simulink model "a_openloop"  (R2022b)
settings: Solver=VariableStepAuto  StartTime=0.0  StopTime=1.0  RelTol=1e-3
libraries: simulink x3, spsDCVoltageSourceLib x1, spsGroundLib x1, spsPermanentMagnetSynchronousMachineLib x1, spsThreePhaseVIMeasurementLib x1, spsUniversalBridgeLib x1, spspowerguiLib x1, sps_lib x1
settings Model: Creator=15403  LastModifiedBy=15403

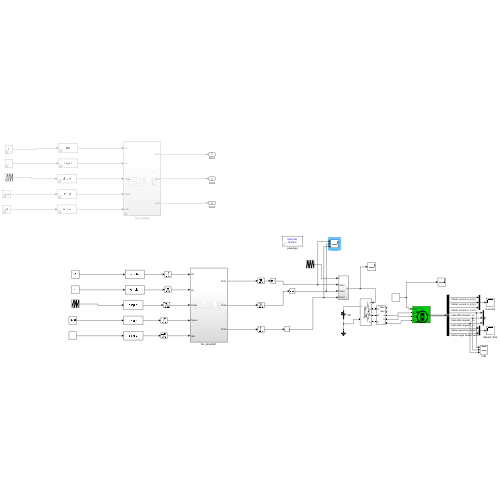
[thumbnail: Simulink's stored preview of the top-level diagram]
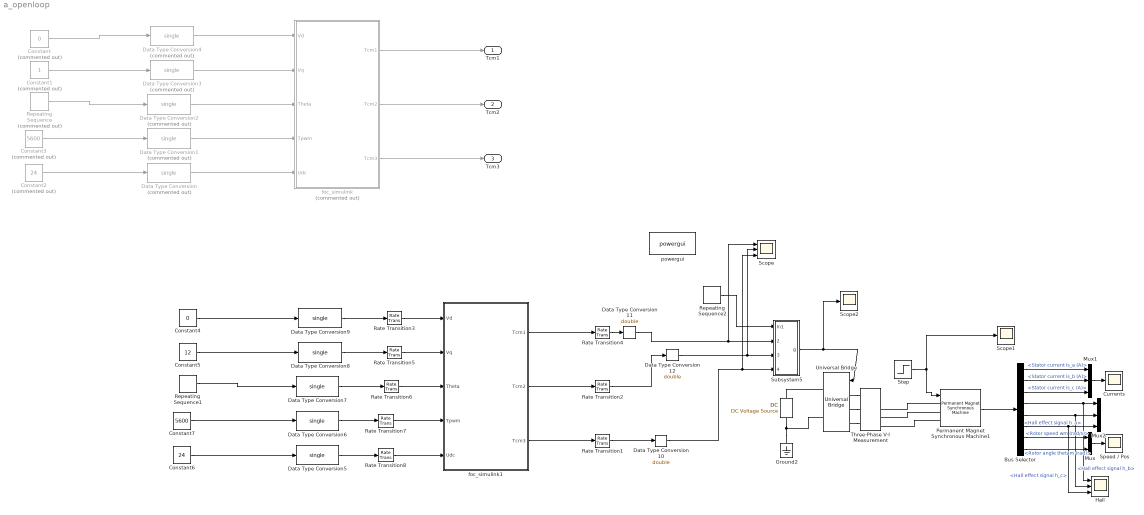
== system a_openloop ==
  Bus Selector : BusSelector  OutputSignals=Stator current is_a (A),Stator current is_b (A),Stator current is_c (A),Hall effect signal h_a,Hall effect signal h_b,Hall effect signal h_c,Rotor speed wm (rad/s),Rotor angle thetam (rad)
  Constant : Constant  Commented=on  Value=0
  Constant1 : Constant  Commented=on
  Constant2 : Constant  Commented=on  Value=24
  Constant3 : Constant  Commented=on  Value=5600
  Constant4 : Constant  Value=0
  Constant5 : Constant  Value=12
  Constant6 : Constant  Value=24
  Constant7 : Constant  Value=5600
  Currents : Scope
  "DC " : spsDCVoltageSourceLib/DC Voltage Source  Amplitude=24  Measurements=None
  Data Type Conversion{,1..4} (5 alike) : DataTypeConversion  Commented=on  OutDataTypeStr=single  SaturateOnIntegerOverflow=off  RndMeth=Floor
  Data Type Conversion10 : DataTypeConversion  OutDataTypeStr=double  SaturateOnIntegerOverflow=off  RndMeth=Floor
  Data Type Conversion11 : DataTypeConversion  OutDataTypeStr=double  SaturateOnIntegerOverflow=off  RndMeth=Floor
  Data Type Conversion12 : DataTypeConversion  OutDataTypeStr=double  SaturateOnIntegerOverflow=off  RndMeth=Floor
  Data Type Conversion{5..9} (5 alike) : DataTypeConversion  OutDataTypeStr=single  SaturateOnIntegerOverflow=off  RndMeth=Floor
  Ground2 : spsGroundLib/Ground  LConnTagsString=a
  Hall : Scope  NumInputPorts=3
  Mux : Mux  Inputs=2
  Mux1 : Mux  Inputs=3
  Mux2 : Mux  Inputs=3
  Permanent Magnet Synchronous Machine1 : spsPermanentMagnetSynchronousMachineLib/Permanent Magnet Synchronous Machine  NbPhases=3  FluxDistribution=Sinusoidal  RotorType=Round  MechanicalLoad=Torque Tm  PresetModel=No  ShowDetailedParameters=on  MeasurementBus=off  Resistance=0.6  Inductance=8.5e-3  dqInductances=[8.5e-3, 8.5e-3]  La=1.4e-3  MachineConstant=Flux linkage established by magnets (V.s)  Flux=0.034182  VoltageCst=6.1999  TorqueCst=0.051273  Flat=120  Mechanical=[1.1e-5,1e-4,1,0.02]  PolePairs=4  InitialConditions=[0,0, 0,0]  InitialConditions5ph=[0 0 0 0 0 0]  RefAngle=Aligned with phase A axis (original Park)  IterativeDiscreteModel=Trapezoidal non iterative  TsBlock=-1  TsPowergui=0
  Rate Transition{1..8} (8 alike) : RateTransition
  Repeating Sequence : simulink/Sources/Repeating Sequence  Commented=on  rep_seq_t=[0 0.1]  rep_seq_y=[0 2 * pi]
  Repeating Sequence1 : simulink/Sources/Repeating Sequence  rep_seq_t=[0 0.1]  rep_seq_y=[0 2 * pi]
  Repeating Sequence2 : simulink/Sources/Repeating Sequence  rep_seq_t=[0 1/15000 2/15000]  rep_seq_y=[0 2800 0]
  Scope : Scope  NumInputPorts=3
  Scope1 : Scope
  Scope2 : Scope
  Speed / Pos : Scope
  Step : Step  Time=0  After=0  SampleTime=0
  Subsystem5 : Subsystem
  Three-Phase V-I Measurement : spsThreePhaseVIMeasurementLib/Three-Phase V-I Measurement  VoltageMeasurement=phase-to-ground  SetLabelV=off  LabelV=Vabc  Vpu=off  VpuLL=off  CurrentMeasurement=yes  SetLabelI=off  LabelI=Iabc  Ipu=off  Pbase=100e6  Vbase=500e3  OutputType=Complex  PhasorSimulation=off  PSBequivalent=0
  Universal Bridge : spsUniversalBridgeLib/Universal Bridge  Arms=3  SnubberResistance=1e5  SnubberCapacitance=inf  Device=IGBT / Diodes  Ron=1e-3  Lon=0  ForwardVoltages="[  0  0  ]"  ForwardVoltage=0  GTOparameters=[ 10e-6 , 20e-6 ]  IGBTparameters=[ 1e-6 , 2e-6 ]  Measurements=None  Measurements_2=None  converterType=Rectifier
  foc_simulink : Subsystem  Commented=on
  foc_simulink1 : Subsystem
  powergui : sps_lib/powergui  Priority=1  SimulationMode=Discrete  SampleTime=0.000001  frequency=60  Iterations=50  frequencyindice=0  Pbase=100e6  ErrMax=1e-4  UnitsV=kV  UnitsW=MW  buscounter=0  FunctionMessages=off  echomessages=off  EnableUseOfTLC=off  CurrentSourceSwitches=off  DisableSnubberDevices=off  DisableRonSwitches=off  DisableVfSwitches=off  DisplayEquations=off  AutomaticDiscreteSolvers=off  SolverType=Tustin/Backward Euler (TBE)  Interpol=off  ExternalGateDelay=off  methode=off  Ts=100  x0status=blocks  SPID=on  SwTol=0  HookPort=off  NonlinearTolerance=1e-4  nMaxIteration=100  ContinueOnMaxIteration=off  RestoreLinks=warning  ResistiveCurrentMeasurement=off  Frange=[0:2:500]  Ylog=off  Xlog=on  ShowGrid=off  save=off  variable=ZData  structure=0  ZoomFFT=off  StartTime=0.0  cycles=1  DisplayStyle=1  fundamental=60  FreqAxis=off  MaxFrequency=1000  frequencyindicesteady=1  RmsSteady=1  display=off
  Tcm1 : Outport
  Tcm2 : Outport  Port=2
  Tcm3 : Outport  Port=3
  wires:
  foc_simulink/3(Tcm3) -> Tcm3/1
  foc_simulink/1(Tcm1) -> Tcm1/1
  Repeating Sequence/1 -> Data Type Conversion2/1
  foc_simulink/2(Tcm2) -> Tcm2/1
  Constant2/1 -> Data Type Conversion/1
  Data Type Conversion3/1 -> foc_simulink/2(Vq)
  Data Type Conversion4/1 -> foc_simulink/1(Vd)
  Constant3/1 -> Data Type Conversion1/1
  Data Type Conversion2/1 -> foc_simulink/3(Theta)
  Data Type Conversion1/1 -> foc_simulink/4(Tpwm)
  Constant/1 -> Data Type Conversion4/1
  Constant1/1 -> Data Type Conversion3/1
  Data Type Conversion/1 -> foc_simulink/5(Udc)
  Rate Transition8/1 -> foc_simulink1/5(Udc)
  Data Type Conversion11/1 -> Scope/1, Subsystem5/2(Tcm1)
  Data Type Conversion12/1 -> Scope/2, Subsystem5/3(Tcm2)
  Bus Selector/6 -> Mux2/3, Hall/3  "<Hall effect signal h_c>"
  Bus Selector/2 -> Mux1/2  "<Stator current is_b (A)>"
  Rate Transition5/1 -> foc_simulink1/2(Vq)
  Rate Transition2/1 -> Data Type Conversion12/1
  Bus Selector/8 -> Mux/2  "<Rotor angle thetam (rad)>"
  Repeating Sequence2/1 -> Subsystem5/1(In1)
  Rate Transition3/1 -> foc_simulink1/1(Vd)
  Permanent Magnet Synchronous Machine1/1 -> Bus Selector/1
  Bus Selector/3 -> Mux1/3  "<Stator current is_c (A)>"
  Step/1 -> Permanent Magnet Synchronous Machine1/1, Scope1/1
  Subsystem5/1(g) -> Scope2/1, Universal Bridge/1
  Mux1/1 -> Currents/1
  Data Type Conversion10/1 -> Subsystem5/4(Tcm3), Scope/3
  Rate Transition1/1 -> Data Type Conversion10/1
  Bus Selector/5 -> Mux2/2, Hall/2  "<Hall effect signal h_b>"
  Repeating Sequence1/1 -> Data Type Conversion7/1
  Rate Transition7/1 -> foc_simulink1/4(Tpwm)
  Constant6/1 -> Data Type Conversion5/1
  Bus Selector/1 -> Mux1/1  "<Stator current is_a (A)>"
  Mux/1 -> Speed / Pos/1
  foc_simulink1/1(Tcm1) -> Rate Transition4/1
  Rate Transition6/1 -> foc_simulink1/3(Theta)
  Bus Selector/4 -> Hall/1, Mux2/1  "<Hall effect signal h_a>"
  Bus Selector/7 -> Mux/1  "<Rotor speed wm (rad/s)>"
  Rate Transition4/1 -> Data Type Conversion11/1
  Data Type Conversion5/1 -> Rate Transition8/1
  Constant5/1 -> Data Type Conversion8/1
  Data Type Conversion9/1 -> Rate Transition3/1
  foc_simulink1/2(Tcm2) -> Rate Transition2/1
  Data Type Conversion8/1 -> Rate Transition5/1
  Constant7/1 -> Data Type Conversion6/1
  Data Type Conversion6/1 -> Rate Transition7/1
  Constant4/1 -> Data Type Conversion9/1
  Data Type Conversion7/1 -> Rate Transition6/1
  foc_simulink1/3(Tcm3) -> Rate Transition1/1
  connections:
  Ground2/LConn1 -- "DC "/LConn1 -- Universal Bridge/RConn2
  Universal Bridge/LConn1 -- Three-Phase V-I Measurement/LConn1
  Permanent Magnet Synchronous Machine1/LConn2 -- Three-Phase V-I Measurement/RConn2
  Universal Bridge/LConn3 -- Three-Phase V-I Measurement/LConn3
  Universal Bridge/LConn2 -- Three-Phase V-I Measurement/LConn2
  Permanent Magnet Synchronous Machine1/LConn1 -- Three-Phase V-I Measurement/RConn1
  "DC "/RConn1 -- Universal Bridge/RConn1
  Permanent Magnet Synchronous Machine1/LConn3 -- Three-Phase V-I Measurement/RConn3

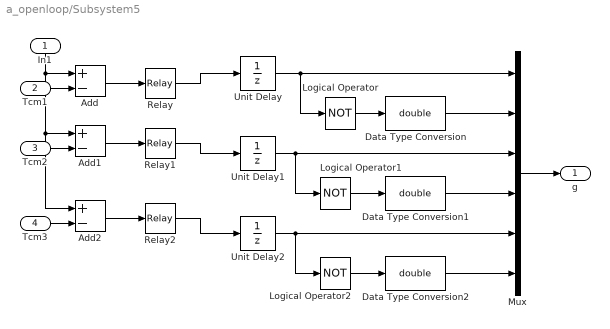
== system a_openloop/Subsystem5 ==
  In1 : Inport
  Tcm1 : Inport  Port=2
  Tcm2 : Inport  Port=3
  Tcm3 : Inport  Port=4
  Add : Sum  Inputs=+-
  Add1 : Sum  Inputs=+-
  Add2 : Sum  Inputs=+-
  Data Type Conversion : DataTypeConversion  OutDataTypeStr=double  SaturateOnIntegerOverflow=off  RndMeth=Floor
  Data Type Conversion1 : DataTypeConversion  OutDataTypeStr=double  SaturateOnIntegerOverflow=off  RndMeth=Floor
  Data Type Conversion2 : DataTypeConversion  OutDataTypeStr=double  SaturateOnIntegerOverflow=off  RndMeth=Floor
  Logical Operator : Logic  Operator=NOT  AllPortsSameDT=off  OutDataTypeStr=boolean
  Logical Operator1 : Logic  Operator=NOT  AllPortsSameDT=off  OutDataTypeStr=boolean
  Logical Operator2 : Logic  Operator=NOT  AllPortsSameDT=off  OutDataTypeStr=boolean
  Mux : Mux  Inputs=6
  Relay : Relay  OffSwitchValue=-eps
  Relay1 : Relay  OffSwitchValue=-eps
  Relay2 : Relay  OffSwitchValue=-eps
  Unit Delay : UnitDelay  SampleTime=-1  HasFrameUpgradeWarning=on
  Unit Delay1 : UnitDelay  SampleTime=-1  HasFrameUpgradeWarning=on
  Unit Delay2 : UnitDelay  SampleTime=-1  HasFrameUpgradeWarning=on
  g : Outport  VectorParamsAs1DForOutWhenUnconnected=off
  wires:
  Tcm3/1 -> Add2/2
  Tcm2/1 -> Add1/2
  Tcm1/1 -> Add/2
  Relay2/1 -> Unit Delay2/1
  Relay1/1 -> Unit Delay1/1
  Relay/1 -> Unit Delay/1
  Unit Delay2/1 -> Mux/5, Logical Operator2/1
  Unit Delay1/1 -> Mux/3, Logical Operator1/1
  Unit Delay/1 -> Logical Operator/1, Mux/1
  Mux/1 -> g/1
  Data Type Conversion/1 -> Mux/2
  Data Type Conversion1/1 -> Mux/4
  Data Type Conversion2/1 -> Mux/6
  Logical Operator2/1 -> Data Type Conversion2/1
  Logical Operator1/1 -> Data Type Conversion1/1
  Logical Operator/1 -> Data Type Conversion/1
  Add1/1 -> Relay1/1
  Add2/1 -> Relay2/1
  Add/1 -> Relay/1
  In1/1 -> Add/1, Add2/1, Add1/1

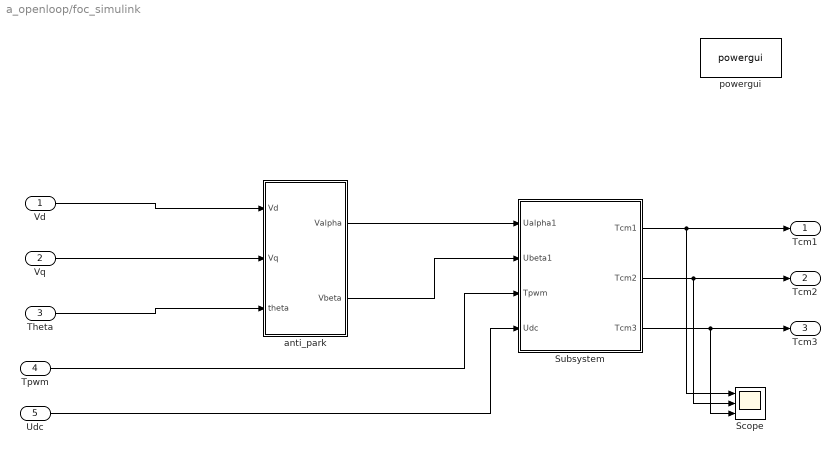
== system a_openloop/foc_simulink ==
  Vd : Inport
  Vq : Inport  Port=2
  Theta : Inport  Port=3
  Tpwm : Inport  Port=4
  Udc : Inport  Port=5
  Scope : Scope  NumInputPorts=3
  Subsystem : Subsystem
  anti_park : Subsystem
  powergui : spspowerguiLib/powergui  Priority=1  SimulationMode=Discrete  SampleTime=50e-6  frequency=60  Iterations=50  frequencyindice=0  Pbase=100e6  ErrMax=1e-4  UnitsV=kV  UnitsW=MW  buscounter=0  FunctionMessages=off  echomessages=off  EnableUseOfTLC=off  CurrentSourceSwitches=off  DisableSnubberDevices=off  DisableRonSwitches=off  DisableVfSwitches=off  DisplayEquations=off  AutomaticDiscreteSolvers=off  SolverType=Tustin/Backward Euler (TBE)  Interpol=off  ExternalGateDelay=off  methode=off  Ts=100  x0status=blocks  SPID=on  SwTol=0  HookPort=off  NonlinearTolerance=1e-4  nMaxIteration=100  ContinueOnMaxIteration=off  RestoreLinks=warning  ResistiveCurrentMeasurement=off  Frange=[0:2:500]  Ylog=off  Xlog=on  ShowGrid=off  save=off  variable=ZData  structure=0  ZoomFFT=off  StartTime=0.0  cycles=1  DisplayStyle=1  fundamental=60  FreqAxis=off  MaxFrequency=1000  frequencyindicesteady=1  RmsSteady=1  display=off
  Tcm1 : Outport
  Tcm2 : Outport  Port=2
  Tcm3 : Outport  Port=3
  wires:
  Vd/1 -> anti_park/1(Vd)
  Theta/1 -> anti_park/3(theta)
  Udc/1 -> Subsystem/4(Udc)
  Tpwm/1 -> Subsystem/3(Tpwm)
  Vq/1 -> anti_park/2(Vq)
  Subsystem/3(Tcm3) -> Scope/3, Tcm3/1
  anti_park/2(Vbeta) -> Subsystem/2(Ubeta1)
  Subsystem/1(Tcm1) -> Scope/1, Tcm1/1
  Subsystem/2(Tcm2) -> Tcm2/1, Scope/2
  anti_park/1(Valpha) -> Subsystem/1(Ualpha1)

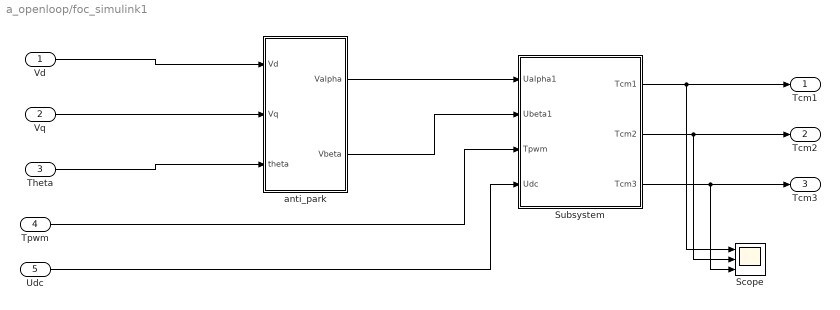
== system a_openloop/foc_simulink1 ==
  Vd : Inport
  Vq : Inport  Port=2
  Theta : Inport  Port=3
  Tpwm : Inport  Port=4
  Udc : Inport  Port=5
  Scope : Scope  NumInputPorts=3
  Subsystem : Subsystem
  anti_park : Subsystem
  Tcm1 : Outport
  Tcm2 : Outport  Port=2
  Tcm3 : Outport  Port=3
  wires:
  Vd/1 -> anti_park/1(Vd)
  Theta/1 -> anti_park/3(theta)
  Udc/1 -> Subsystem/4(Udc)
  Tpwm/1 -> Subsystem/3(Tpwm)
  Vq/1 -> anti_park/2(Vq)
  Subsystem/3(Tcm3) -> Scope/3, Tcm3/1
  anti_park/2(Vbeta) -> Subsystem/2(Ubeta1)
  Subsystem/1(Tcm1) -> Scope/1, Tcm1/1
  Subsystem/2(Tcm2) -> Tcm2/1, Scope/2
  anti_park/1(Valpha) -> Subsystem/1(Ualpha1)

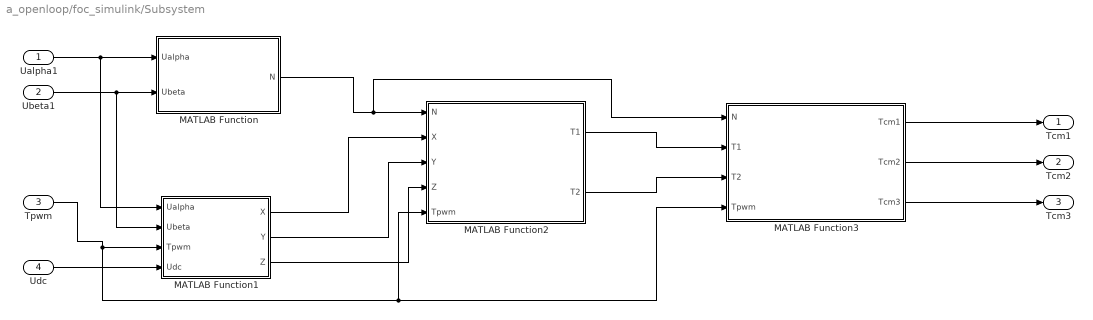
== system a_openloop/foc_simulink/Subsystem ==
  Ualpha1 : Inport
  Ubeta1 : Inport  Port=2
  Tpwm : Inport  Port=3
  Udc : Inport  Port=4
  MATLAB Function : MATLAB Function  TreatAsAtomicUnit=on
  MATLAB Function1 : MATLAB Function  TreatAsAtomicUnit=on
  MATLAB Function2 : MATLAB Function  TreatAsAtomicUnit=on
  MATLAB Function3 : MATLAB Function  TreatAsAtomicUnit=on
  Tcm1 : Outport
  Tcm2 : Outport  Port=2
  Tcm3 : Outport  Port=3
  wires:
  MATLAB Function3/2(Tcm2) -> Tcm2/1
  Tpwm/1 -> MATLAB Function3/4(Tpwm), MATLAB Function2/5(Tpwm), MATLAB Function1/3(Tpwm)
  MATLAB Function/1(N) -> MATLAB Function3/1(N), MATLAB Function2/1(N)
  Udc/1 -> MATLAB Function1/4(Udc)
  MATLAB Function3/3(Tcm3) -> Tcm3/1
  MATLAB Function2/1(T1) -> MATLAB Function3/2(T1)
  Ualpha1/1 -> MATLAB Function1/1(Ualpha), MATLAB Function/1(Ualpha)
  MATLAB Function2/2(T2) -> MATLAB Function3/3(T2)
  Ubeta1/1 -> MATLAB Function1/2(Ubeta), MATLAB Function/2(Ubeta)
  MATLAB Function3/1(Tcm1) -> Tcm1/1
  MATLAB Function1/1(X) -> MATLAB Function2/2(X)
  MATLAB Function1/3(Z) -> MATLAB Function2/4(Z)
  MATLAB Function1/2(Y) -> MATLAB Function2/3(Y)

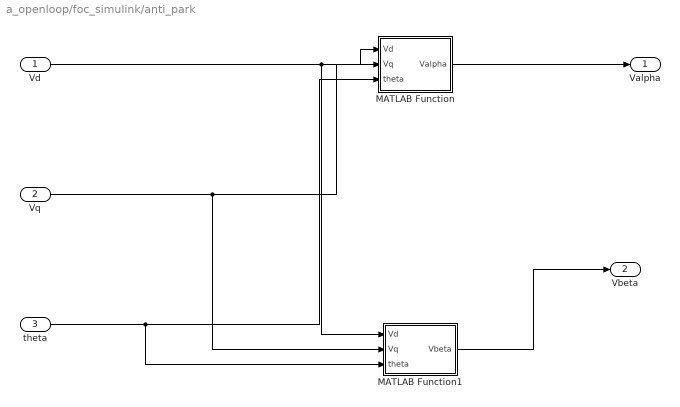
== system a_openloop/foc_simulink/anti_park ==
  Vd : Inport
  Vq : Inport  Port=2
  theta : Inport  Port=3
  MATLAB Function : MATLAB Function  TreatAsAtomicUnit=on
  MATLAB Function1 : MATLAB Function  TreatAsAtomicUnit=on
  Valpha : Outport
  Vbeta : Outport  Port=2
  wires:
  MATLAB Function/1(Valpha) -> Valpha/1
  MATLAB Function1/1(Vbeta) -> Vbeta/1
  Vd/1 -> MATLAB Function/1(Vd), MATLAB Function1/1(Vd)
  Vq/1 -> MATLAB Function/2(Vq), MATLAB Function1/2(Vq)
  theta/1 -> MATLAB Function/3(theta), MATLAB Function1/3(theta)

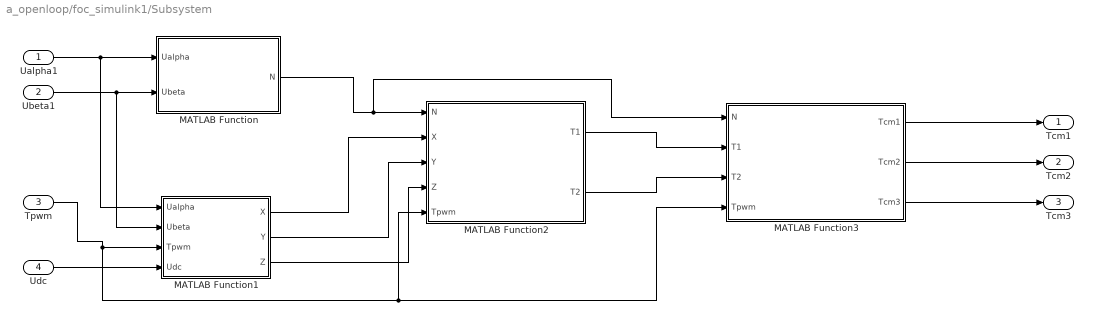
== system a_openloop/foc_simulink1/Subsystem ==
  Ualpha1 : Inport
  Ubeta1 : Inport  Port=2
  Tpwm : Inport  Port=3
  Udc : Inport  Port=4
  MATLAB Function : MATLAB Function  TreatAsAtomicUnit=on
  MATLAB Function1 : MATLAB Function  TreatAsAtomicUnit=on
  MATLAB Function2 : MATLAB Function  TreatAsAtomicUnit=on
  MATLAB Function3 : MATLAB Function  TreatAsAtomicUnit=on
  Tcm1 : Outport
  Tcm2 : Outport  Port=2
  Tcm3 : Outport  Port=3
  wires:
  MATLAB Function3/2(Tcm2) -> Tcm2/1
  Tpwm/1 -> MATLAB Function3/4(Tpwm), MATLAB Function2/5(Tpwm), MATLAB Function1/3(Tpwm)
  MATLAB Function/1(N) -> MATLAB Function3/1(N), MATLAB Function2/1(N)
  Udc/1 -> MATLAB Function1/4(Udc)
  MATLAB Function3/3(Tcm3) -> Tcm3/1
  MATLAB Function2/1(T1) -> MATLAB Function3/2(T1)
  Ualpha1/1 -> MATLAB Function1/1(Ualpha), MATLAB Function/1(Ualpha)
  MATLAB Function2/2(T2) -> MATLAB Function3/3(T2)
  Ubeta1/1 -> MATLAB Function1/2(Ubeta), MATLAB Function/2(Ubeta)
  MATLAB Function3/1(Tcm1) -> Tcm1/1
  MATLAB Function1/1(X) -> MATLAB Function2/2(X)
  MATLAB Function1/3(Z) -> MATLAB Function2/4(Z)
  MATLAB Function1/2(Y) -> MATLAB Function2/3(Y)

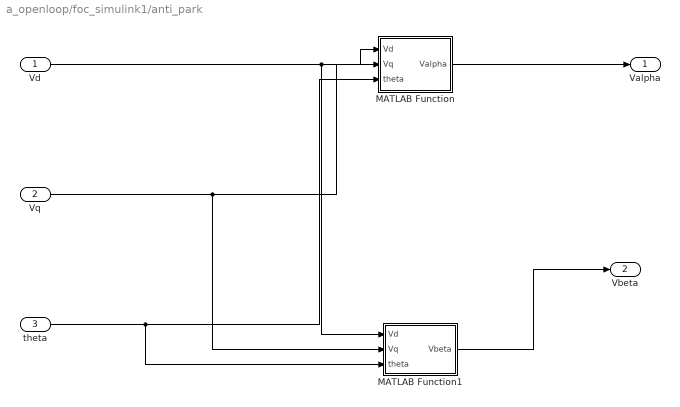
== system a_openloop/foc_simulink1/anti_park ==
  Vd : Inport
  Vq : Inport  Port=2
  theta : Inport  Port=3
  MATLAB Function : MATLAB Function  TreatAsAtomicUnit=on
  MATLAB Function1 : MATLAB Function  TreatAsAtomicUnit=on
  Valpha : Outport
  Vbeta : Outport  Port=2
  wires:
  MATLAB Function/1(Valpha) -> Valpha/1
  MATLAB Function1/1(Vbeta) -> Vbeta/1
  Vd/1 -> MATLAB Function/1(Vd), MATLAB Function1/1(Vd)
  Vq/1 -> MATLAB Function/2(Vq), MATLAB Function1/2(Vq)
  theta/1 -> MATLAB Function/3(theta), MATLAB Function1/3(theta)

== matlab function a_openloop/foc_simulink/Subsystem/MATLAB Function1 ==
  data: Ualpha input; Ubeta input; Tpwm input; Udc input; X output; Y output; Z output
function [X, Y, Z] = fcn(Ualpha, Ubeta, Tpwm, Udc)

X = sqrt(3) * Tpwm * Ubeta / Udc;
Y = sqrt(3) * Tpwm / Udc * (sqrt(3) / 2 * Ualpha + 1 / 2 * Ubeta);
Z = sqrt(3) * Tpwm / Udc * (-sqrt(3) / 2 * Ualpha + 1 / 2 * Ubeta);

== matlab function a_openloop/foc_simulink/Subsystem/MATLAB Function2 ==
  data: N input; T1 output; X input; Y input; Z input; Tpwm input; T2 output
function [T1, T2] = fcn(N, X, Y, Z, Tpwm)

T1 = single(0);
T2 = single(0);

if N == 1
    T1 = Z;
    T2 = Y;
elseif N == 2
    T1 = Y;
    T2 = -X;
elseif N == 3
    T1 = -Z;
    T2 = X;
elseif N == 4
    T1 = -X;
    T2 = Z;
elseif N == 5
    T1 = X;
    T2 = -Y;
elseif N == 6
    T1 = -Y;
    T2 = -Z;
end

== matlab function a_openloop/foc_simulink/Subsystem/MATLAB Function3 ==
  data: N input; Tcm1 output; T1 input; T2 input; Tpwm input; Tcm2 output; Tcm3 output
function [Tcm1, Tcm2, Tcm3] = fcn(N, T1, T2, Tpwm)

Tcm1 = single(0);
Tcm2 = single(0);
Tcm3 = single(0);


if N == 1
    Tcm1 = (Tpwm + T1 - T2) / 4;
    Tcm2 = (Tpwm - T1 - T2) / 4;
    Tcm3 = (Tpwm + T1 + T2) / 4;
elseif N == 2
    Tcm1 = (Tpwm - T1 - T2) / 4;
    Tcm2 = (Tpwm + T1 + T2) / 4;
    Tcm3 = (Tpwm + T1 - T2) / 4;
elseif N == 3
    Tcm1 = (Tpwm - T1 - T2) / 4;
    Tcm2 = (Tpwm + T1 - T2) / 4;
    Tcm3 = (Tpwm + T1 + T2) / 4;
elseif N == 4
    Tcm1 = (Tpwm + T1 + T2) / 4;
    Tcm2 = (Tpwm + T1 - T2) / 4;
    Tcm3 = (Tpwm - T1 - T2) / 4;
elseif N == 5
    Tcm1 = (Tpwm + T1 + T2) / 4;
    Tcm2 = (Tpwm - T1 - T2) / 4;
    Tcm3 = (Tpwm + T1 - T2) / 4;
elseif N == 6
    Tcm1 = (Tpwm + T1 - T2) / 4;
    Tcm2 = (Tpwm + T1 + T2) / 4;
    Tcm3 = (Tpwm - T1 - T2) / 4;
end

== matlab function a_openloop/foc_simulink/anti_park/MATLAB Function1 ==
  data: Vd input; Vbeta output; Vq input; theta input
function Vbeta = fcn(Vd, Vq, theta)

Vbeta = Vd * sin(theta) + Vq * cos(theta);

== matlab function a_openloop/foc_simulink/anti_park/MATLAB Function ==
  data: Vd input; Valpha output; Vq input; theta input
function Valpha = fcn(Vd, Vq, theta)

Valpha = Vd * cos(theta) - Vq * sin(theta);

== matlab function a_openloop/foc_simulink1/Subsystem/MATLAB Function ==
  data: Ualpha input; N output; Ubeta input
function N = fcn(Ualpha, Ubeta)

U1 = Ubeta;
U2 = sqrt(3) * Ualpha - Ubeta;
U3 = -sqrt(3) * Ualpha - Ubeta;
A = 0;
B = 0;
C = 0;

if U1 > 0
    A = 1;
else
    A = 0;
end

if U2 > 0
    B = 1;
else
    B = 0;
end

if U3 > 0
    C = 1;
else
    C = 0;
end

N = A + 2 * B + 4 * C;

== matlab function a_openloop/foc_simulink1/Subsystem/MATLAB Function1 ==
  data: Ualpha input; Ubeta input; Tpwm input; Udc input; X output; Y output; Z output
function [X, Y, Z] = fcn(Ualpha, Ubeta, Tpwm, Udc)

X = sqrt(3) * Tpwm * Ubeta / Udc;
Y = sqrt(3) * Tpwm / Udc * (sqrt(3) / 2 * Ualpha + 1 / 2 * Ubeta);
Z = sqrt(3) * Tpwm / Udc * (-sqrt(3) / 2 * Ualpha + 1 / 2 * Ubeta);

== matlab function a_openloop/foc_simulink1/Subsystem/MATLAB Function2 ==
  data: N input; T1 output; X input; Y input; Z input; Tpwm input; T2 output
function [T1, T2] = fcn(N, X, Y, Z, Tpwm)

T1 = single(0);
T2 = single(0);

if N == 1
    T1 = Z;
    T2 = Y;
elseif N == 2
    T1 = Y;
    T2 = -X;
elseif N == 3
    T1 = -Z;
    T2 = X;
elseif N == 4
    T1 = -X;
    T2 = Z;
elseif N == 5
    T1 = X;
    T2 = -Y;
elseif N == 6
    T1 = -Y;
    T2 = -Z;
end

== matlab function a_openloop/foc_simulink1/Subsystem/MATLAB Function3 ==
  data: N input; Tcm1 output; T1 input; T2 input; Tpwm input; Tcm2 output; Tcm3 output
function [Tcm1, Tcm2, Tcm3] = fcn(N, T1, T2, Tpwm)

Tcm1 = single(0);
Tcm2 = single(0);
Tcm3 = single(0);


if N == 1
    Tcm1 = (Tpwm + T1 - T2) / 4;
    Tcm2 = (Tpwm - T1 - T2) / 4;
    Tcm3 = (Tpwm + T1 + T2) / 4;
elseif N == 2
    Tcm1 = (Tpwm - T1 - T2) / 4;
    Tcm2 = (Tpwm + T1 + T2) / 4;
    Tcm3 = (Tpwm + T1 - T2) / 4;
elseif N == 3
    Tcm1 = (Tpwm - T1 - T2) / 4;
    Tcm2 = (Tpwm + T1 - T2) / 4;
    Tcm3 = (Tpwm + T1 + T2) / 4;
elseif N == 4
    Tcm1 = (Tpwm + T1 + T2) / 4;
    Tcm2 = (Tpwm + T1 - T2) / 4;
    Tcm3 = (Tpwm - T1 - T2) / 4;
elseif N == 5
    Tcm1 = (Tpwm + T1 + T2) / 4;
    Tcm2 = (Tpwm - T1 - T2) / 4;
    Tcm3 = (Tpwm + T1 - T2) / 4;
elseif N == 6
    Tcm1 = (Tpwm + T1 - T2) / 4;
    Tcm2 = (Tpwm + T1 + T2) / 4;
    Tcm3 = (Tpwm - T1 - T2) / 4;
end

== matlab function a_openloop/foc_simulink1/anti_park/MATLAB Function ==
  data: Vd input; Valpha output; Vq input; theta input
function Valpha = fcn(Vd, Vq, theta)

Valpha = Vd * cos(theta) - Vq * sin(theta);

== matlab function a_openloop/foc_simulink1/anti_park/MATLAB Function1 ==
  data: Vd input; Vbeta output; Vq input; theta input
function Vbeta = fcn(Vd, Vq, theta)

Vbeta = Vd * sin(theta) + Vq * cos(theta);

== matlab function a_openloop/foc_simulink/Subsystem/MATLAB Function ==
  data: Ualpha input; N output; Ubeta input
function N = fcn(Ualpha, Ubeta)

U1 = Ubeta;
U2 = sqrt(3) * Ualpha - Ubeta;
U3 = -sqrt(3) * Ualpha - Ubeta;
A = 0;
B = 0;
C = 0;

if U1 > 0
    A = 1;
else
    A = 0;
end

if U2 > 0
    B = 1;
else
    B = 0;
end

if U3 > 0
    C = 1;
else
    C = 0;
end

N = A + 2 * B + 4 * C;
